simulink model "Tomato_Crop_Control_Main"  (R2025b)
settings: Solver=FixedStepDiscrete  StartTime=0  StopTime=24  FixedStep=0.01  RelTol=1e-3
model workspace (MAT data in the model file):
  Ts = 0.01
  ctrlType = 3
  sensorNoise.time = [0 0.01 0.02 0.03 0.04 0.05 0.06 0.07 0.08 0.09 0.1 0.11 ... (2401 elements, 2401x1)]
  sensorNoise.signals.values = [0.144198042187 -0.535824758394 0.0585721764367 0.102054484425 0.0457535498354 -0.621619945954 0.0176579908891 -0.0995075158765 0.168146871715 0.298844225523 0.375893759453 0.190077020908 ... (26411 elements, 2401x11)]
  sensorNoise.signals.dimensions = 11
  x0 = [60; 25; 65; 15000; 6.35; 2.4; 130; 48; 180; 80; 100]
settings Model: Creator=abhi8  LastModifiedBy=abhi8

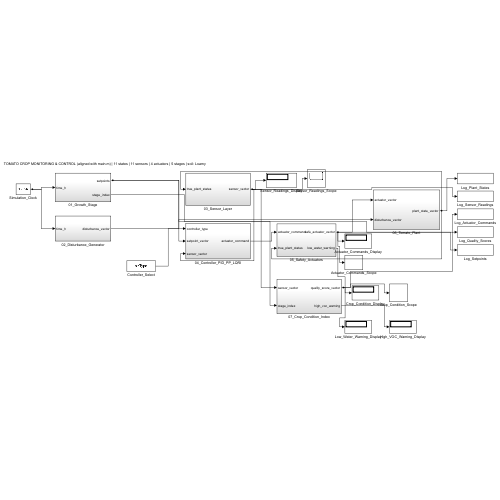
[thumbnail: Simulink's stored preview of the top-level diagram]
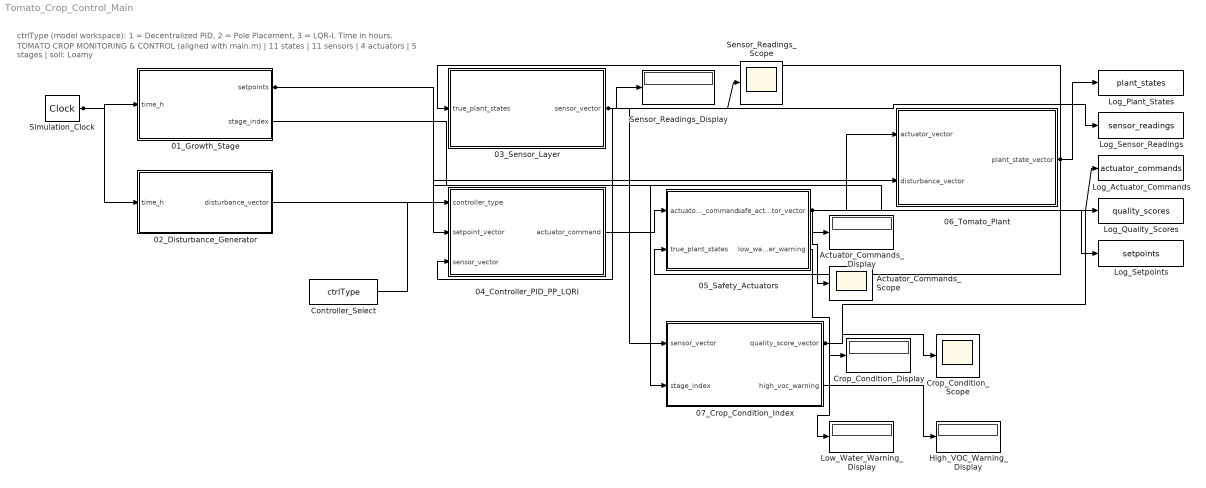
== system Tomato_Crop_Control_Main ==
  note: TOMATO CROP MONITORING & CONTROL (aligned with main.m) | 11 states | 11 sensors | 4 actuators | 5 stages | soil: Loamy
  note: ctrlType (model workspace): 1 = Decentralized PID, 2 = Pole Placement, 3 = LQR-I. Time in hours.
  01_Growth_Stage : Subsystem
  02_Disturbance_Generator : Subsystem
  03_Sensor_Layer : Subsystem
  04_Controller_PID_PP_LQRI : Subsystem
  05_Safety_Actuators : Subsystem
  06_Tomato_Plant : Subsystem
  07_Crop_Condition_Index : Subsystem
  Actuator_Commands_Display : Display
  Actuator_Commands_Scope : Scope
  Controller_Select : Constant  Value=ctrlType  SampleTime=Ts
  Crop_Condition_Display : Display
  Crop_Condition_Scope : Scope
  High_VOC_Warning_Display : Display
  Log_Actuator_Commands : ToWorkspace  VariableName=actuator_commands  SaveFormat=Timeseries  SampleTime=-1
  Log_Plant_States : ToWorkspace  VariableName=plant_states  SaveFormat=Timeseries  SampleTime=-1
  Log_Quality_Scores : ToWorkspace  VariableName=quality_scores  SaveFormat=Timeseries  SampleTime=-1
  Log_Sensor_Readings : ToWorkspace  VariableName=sensor_readings  SaveFormat=Timeseries  SampleTime=-1
  Log_Setpoints : ToWorkspace  VariableName=setpoints  SaveFormat=Timeseries  SampleTime=-1
  Low_Water_Warning_Display : Display
  Sensor_Readings_Display : Display
  Sensor_Readings_Scope : Scope
  Simulation_Clock : DigitalClock  SampleTime=Ts
  wires:
  Simulation_Clock/1 -> 01_Growth_Stage/1(time_h), 02_Disturbance_Generator/1(time_h)
  06_Tomato_Plant/1(plant_state_vector) -> 03_Sensor_Layer/1(true_plant_states), 05_Safety_Actuators/2(true_plant_states), Log_Plant_States/1
  Controller_Select/1 -> 04_Controller_PID_PP_LQRI/1(controller_type)
  01_Growth_Stage/1(setpoints) -> 04_Controller_PID_PP_LQRI/2(setpoint_vector), Log_Setpoints/1
  03_Sensor_Layer/1(sensor_vector) -> 04_Controller_PID_PP_LQRI/3(sensor_vector), 07_Crop_Condition_Index/1(sensor_vector), Sensor_Readings_Display/1, Sensor_Readings_Scope/1, Log_Sensor_Readings/1
  04_Controller_PID_PP_LQRI/1(actuator_command) -> 05_Safety_Actuators/1(actuator_command)
  05_Safety_Actuators/1(safe_actuator_vector) -> 06_Tomato_Plant/1(actuator_vector), Actuator_Commands_Display/1, Actuator_Commands_Scope/1, Log_Actuator_Commands/1
  02_Disturbance_Generator/1(disturbance_vector) -> 06_Tomato_Plant/2(disturbance_vector)
  01_Growth_Stage/2(stage_index) -> 07_Crop_Condition_Index/2(stage_index)
  07_Crop_Condition_Index/1(quality_score_vector) -> Crop_Condition_Display/1, Crop_Condition_Scope/1, Log_Quality_Scores/1
  05_Safety_Actuators/2(low_water_warning) -> Low_Water_Warning_Display/1
  07_Crop_Condition_Index/2(high_voc_warning) -> High_VOC_Warning_Display/1

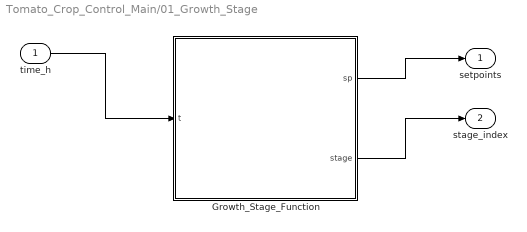
== system Tomato_Crop_Control_Main/01_Growth_Stage ==
  time_h : Inport
  Growth_Stage_Function : MATLAB Function  TreatAsAtomicUnit=on
  setpoints : Outport
  stage_index : Outport  Port=2
  wires:
  time_h/1 -> Growth_Stage_Function/1(t)
  Growth_Stage_Function/1(sp) -> setpoints/1
  Growth_Stage_Function/2(stage) -> stage_index/1

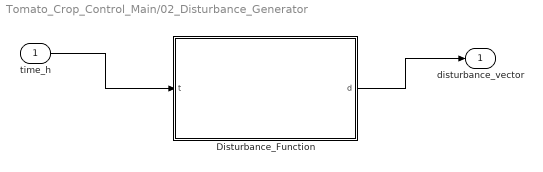
== system Tomato_Crop_Control_Main/02_Disturbance_Generator ==
  time_h : Inport
  Disturbance_Function : MATLAB Function  TreatAsAtomicUnit=on
  disturbance_vector : Outport
  wires:
  time_h/1 -> Disturbance_Function/1(t)
  Disturbance_Function/1(d) -> disturbance_vector/1

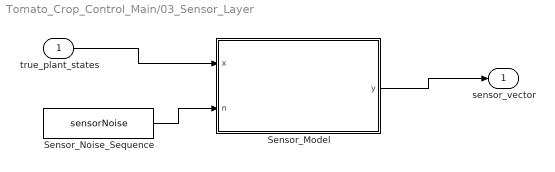
== system Tomato_Crop_Control_Main/03_Sensor_Layer ==
  true_plant_states : Inport
  Sensor_Model : MATLAB Function  TreatAsAtomicUnit=on
  Sensor_Noise_Sequence : FromWorkspace  VariableName=sensorNoise  SampleTime=Ts  Interpolate=off  OutputAfterFinalValue=Holding final value
  sensor_vector : Outport
  wires:
  true_plant_states/1 -> Sensor_Model/1(x)
  Sensor_Noise_Sequence/1 -> Sensor_Model/2(n)
  Sensor_Model/1(y) -> sensor_vector/1

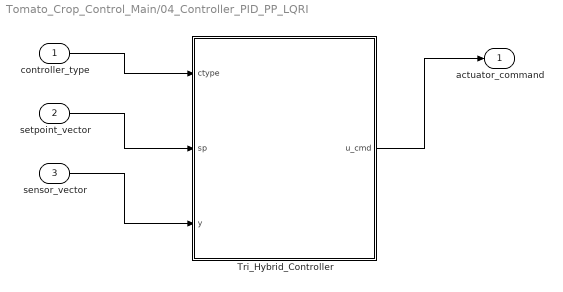
== system Tomato_Crop_Control_Main/04_Controller_PID_PP_LQRI ==
  controller_type : Inport
  setpoint_vector : Inport  Port=2
  sensor_vector : Inport  Port=3
  Tri_Hybrid_Controller : MATLAB Function  TreatAsAtomicUnit=on
  actuator_command : Outport
  wires:
  controller_type/1 -> Tri_Hybrid_Controller/1(ctype)
  setpoint_vector/1 -> Tri_Hybrid_Controller/2(sp)
  sensor_vector/1 -> Tri_Hybrid_Controller/3(y)
  Tri_Hybrid_Controller/1(u_cmd) -> actuator_command/1

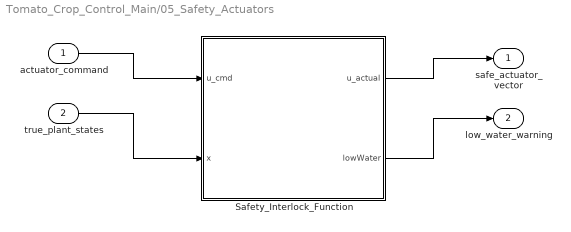
== system Tomato_Crop_Control_Main/05_Safety_Actuators ==
  actuator_command : Inport
  true_plant_states : Inport  Port=2
  Safety_Interlock_Function : MATLAB Function  TreatAsAtomicUnit=on
  safe_actuator_vector : Outport
  low_water_warning : Outport  Port=2
  wires:
  actuator_command/1 -> Safety_Interlock_Function/1(u_cmd)
  true_plant_states/1 -> Safety_Interlock_Function/2(x)
  Safety_Interlock_Function/1(u_actual) -> safe_actuator_vector/1
  Safety_Interlock_Function/2(lowWater) -> low_water_warning/1

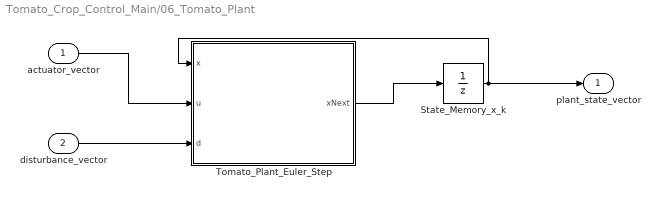
== system Tomato_Crop_Control_Main/06_Tomato_Plant ==
  actuator_vector : Inport
  disturbance_vector : Inport  Port=2
  State_Memory_x_k : UnitDelay  InitialCondition=x0  SampleTime=0.01  HasFrameUpgradeWarning=on
  Tomato_Plant_Euler_Step : MATLAB Function  TreatAsAtomicUnit=on
  plant_state_vector : Outport
  wires:
  State_Memory_x_k/1 -> Tomato_Plant_Euler_Step/1(x), plant_state_vector/1
  actuator_vector/1 -> Tomato_Plant_Euler_Step/2(u)
  disturbance_vector/1 -> Tomato_Plant_Euler_Step/3(d)
  Tomato_Plant_Euler_Step/1(xNext) -> State_Memory_x_k/1

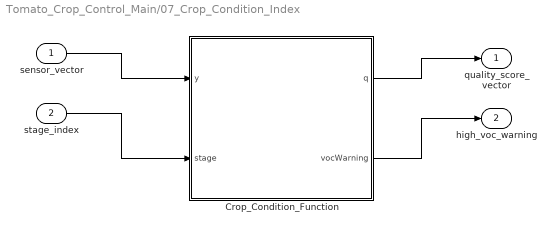
== system Tomato_Crop_Control_Main/07_Crop_Condition_Index ==
  sensor_vector : Inport
  stage_index : Inport  Port=2
  Crop_Condition_Function : MATLAB Function  TreatAsAtomicUnit=on
  quality_score_vector : Outport
  high_voc_warning : Outport  Port=2
  wires:
  sensor_vector/1 -> Crop_Condition_Function/1(y)
  stage_index/1 -> Crop_Condition_Function/2(stage)
  Crop_Condition_Function/1(q) -> quality_score_vector/1
  Crop_Condition_Function/2(vocWarning) -> high_voc_warning/1

== matlab function Tomato_Crop_Control_Main/01_Growth_Stage/Growth_Stage_Function ==
  data: t input; sp output; stage output
function [sp, stage] = GrowthStage(t)
% sp = [moisture; temperature; humidity; light] (main.m db.phase setpoints)
if t < 2
    stage = 1; sp = [70;24;72.5;10000];
elseif t < 8
    stage = 2; sp = [60;25;65;18000];
elseif t < 12
    stage = 3; sp = [58;23.5;62.5;22500];
elseif t < 18
    stage = 4; sp = [65;25;60;22500];
else
    stage = 5; sp = [55;22.5;55;20000];
end
end

== matlab function Tomato_Crop_Control_Main/03_Sensor_Layer/Sensor_Model ==
  data: x input; y output; n input
function y = SensorModel(x, n)
% main.m simulateSensorLayerLocal: y = sat(x + sigma*randn), randn sequence fed in as n
lo = [0;-40;0;0;0;0;0;0;0;0;0];
hi = [100;85;100;65535;14;10;1999;1999;1999;100;500];
noiseOn = 1;
y = zeros(11, 1);
for i = 1:11
    sensed = x(i) + noiseOn * n(i);
    y(i) = max(lo(i), min(hi(i), sensed));
end
end

== matlab function Tomato_Crop_Control_Main/04_Controller_PID_PP_LQRI/Tri_Hybrid_Controller ==
  data: ctype input; u_cmd output; sp input; y input
function u_cmd = TriHybridController(ctype, sp, y)
% ctype: 1 = Decentralized PID, 2 = Pole Placement, 3 = LQR-I (main.m step 6 switch)
persistent intg pe z_int
dt = 0.01;
Kp = [0.080000000000000002;0.20000000000000001;0.10000000000000001;5.0000000000000002e-05];
Ki = [0.014999999999999999;0.02;0.014999999999999999;1.0000000000000001e-05];
Kd = [0.0050000000000000001;0.01;0.0050000000000000001;1.0000000000000001e-05];
u0 = [0.14999999999999999;0.40000000000000008;0.20000000000000004;0];
x0t = [60;25;65;15000;6.3569767441860456;3.0961538461538458;132.14617940199335;53.157370517928278;193.97515527950313;80;100];
Kpp = [0.048333333337184523 -0.00049572649547191604 0 -1.2803268095182857e-08 0 0 0 0 0 0 0;0 -0.21666666660225375 -2.7755575615628914e-17 -1.6507937872024044e-05 0 0 0 0 0 0 0;0 -0.14713541663468468 0.12499999999987499 -1.0615080242334755e-05 0 0 0 0 0 0 0;0 0 0 2.3333327691070732e-05 0 0 0 0 0 0 0];
Kx = [0.33045903239628471 -0.00041190708390725835 1.709435974051306e-05 -2.3561558211869358e-09 -0.00048730567058277003 1.1042346765690718e-05 -4.82261767063196e-07 2.5341090944660356e-06 2.1422647797648958e-06 -2.3389542716528394e-06 7.5156450631499362e-18;0.00012071812895227755 -0.9851642748800985 -0.059883029409090759 -2.6221558787539299e-06 8.2842246792511105e-08 -7.0757158985011595e-06 2.1496635984296123e-07 5.9632600152445188e-07 1.8759197603930526e-07 2.8607042231626474e-09 5.2040316388700277e-21;1.1217806681167034e-05 -0.37126976109372778 0.37426516788265268 -7.6341153907015784e-07 4.7389129263811032e-08 -1.7494050334136512e-06 4.6254791841818205e-08 1.2806484979807713e-07 4.019131706525666e-08 8.3160193500875327e-10 6.8202143908703237e-22;-5.8631339014747203e-06 0.046489321360276642 -0.0053677373840816762 0.00039002337891379279 -1.5258171556508284e-07 4.4013012272865192e-07 -9.19215082032534e-07 -2.6187991014429883e-06 -8.0551413105558905e-07 -8.7458293397006619e-10 -5.1872422376848302e-21];
Kz = [0.63245550435268716 0.0004211622899643958 4.0740750688245492e-05 -7.1243543416210205e-09;0.00020984406328235648 -1.5711911017241582 -0.17357717814678505 4.4155060562703391e-05;6.030330919642846e-06 -0.39163748120451147 0.55605516599390314 2.0221198342119552e-05;-4.6424572517600495e-06 0.097211657880012514 -0.0078367674724567678 0.0012232370229141166];
if isempty(intg),  intg  = zeros(4, 1); end
if isempty(pe),    pe    = zeros(4, 1); end
if isempty(z_int), z_int = zeros(4, 1); end
yv = y(:); spv = sp(:);
u_cmd = zeros(4, 1);
% tracking errors from SENSED values (temperature reversed: fan cools)
e = [spv(1) - yv(1); yv(2) - spv(2); spv(3) - yv(3); spv(4) - yv(4)];
xtarget = x0t; xtarget(1:4) = spv;
if ctype == 1
    for j = 1:4
        ur = Kp(j)*e(j) + Ki(j)*intg(j) + Kd(j)*(e(j) - pe(j))/dt;
        u_cmd(j) = max(0, min(1, ur));
        if ~((ur >= 1 && e(j) > 0) || (ur <= 0 && e(j) < 0))
            intg(j) = intg(j) + e(j) * dt;
        end
        pe(j) = e(j);
    end
elseif ctype == 2
    u_cmd = u0 - Kpp * (yv - xtarget);
else
    u_raw = u0 - Kx * (yv - xtarget) - Kz * z_int;
    u_cmd = max(0, min(1, u_raw));
    y_err = yv(1:4) - spv(1:4);
    for j = 1:4
        push = -Kz(j,j) * y_err(j);
        if ~((u_raw(j) >= 1 && push > 0) || (u_raw(j) <= 0 && push < 0))
            z_int(j) = z_int(j) + y_err(j) * dt;
        end
    end
end
end

== matlab function Tomato_Crop_Control_Main/05_Safety_Actuators/Safety_Interlock_Function ==
  data: u_cmd input; u_actual output; x input; lowWater output
function [u_actual, lowWater] = SafetyLogic(u_cmd, x)
% main.m: actuator saturation, then pump cut-off when TRUE tank level < minimum
u_actual = max(0.0, min(1.0, u_cmd(:)));
lowWater = double(x(10) < 10);
if lowWater > 0
    u_actual(1) = 0.0;
end
end

== matlab function Tomato_Crop_Control_Main/06_Tomato_Plant/Tomato_Plant_Euler_Step ==
  data: x input; u input; xNext output; d input
function xNext = TomatoPlantStep(x, u, d)
% main.m Tomato_Dynamics + forward Euler + enforcePhysicalBoundsLocal
% Soil type: Loamy
dt = 0.01;
minWater = 10;
drainageGain = 0.02; irrigationGain = 12; evapFactor = 2;
drainageThreshold = 50; leachFac = 1;
xv = x(:);
pump      = max(0, min(1, u(1)));
fan       = max(0, min(1, u(2)));
mist      = max(0, min(1, u(3)));
growLight = max(0, min(1, u(4)));
if xv(10) < minWater
    pump = 0.0;
end
extT = d(1); natL = d(2); evap = d(3);
M = xv(1); T = xv(2); L = xv(4); pH = xv(5); EC = xv(6);
N = xv(7); P = xv(8); K = xv(9); VOC = xv(11);
drainage = drainageGain * max(M - drainageThreshold, 0);
moistureLoss = evapFactor * evap * (1 + 0.01 * max(T - 25, 0));
dM = irrigationGain * pump - moistureLoss - drainage;
dT = 0.15 * (extT - T) + 0.00008 * L - 3.0 * fan;
dH = 8.0 * mist - 4.0 * fan - 0.15 * max(T - 25, 0);
dL = 0.5 * (natL - L) + 30000.0 * growLight;
transpiration = (0.50 + 0.50 * (L / 25000.0)) * (1.0 + 0.02 * max(T - 22, 0));
dpH = 0.04 * (6.35 - pH) + 0.02 * (6.45 - pH) * pump - 0.0002 * max(N - 140, 0);
dEC = 0.55 * pump - 0.05 * (evap / 0.8) - 0.03 * leachFac * drainage * EC + 0.02 * (2.4 - EC);
dN = 22.0 * pump - 3.8 * transpiration - 0.05 * leachFac * drainage * (N / 100.0) + 0.03 * (130.0 - N);
dP = 7.5 * pump - 1.2 * transpiration - 0.02 * leachFac * drainage * (P / 50.0) + 0.02 * (48.0 - P);
dK = 28.0 * pump - 4.8 * transpiration - 0.04 * leachFac * drainage * (K / 150.0) + 0.03 * (190.0 - K);
refillNominal = 0.5 * evap + 0.2 * 0.15;
q_refill = 0.05 * (80.0 - xv(10)) + refillNominal;
dWater = q_refill - (0.5 * evap + 0.2 * pump);
dVOC = 0.05 * (100.0 - VOC) + 0.10 * max(T - 30, 0);
dx = [dM; dT; dH; dL; dpH; dEC; dN; dP; dK; dWater; dVOC];
xNext = xv + dx * dt;
lo = [0; -10; 0; 0; 0; 0; 0; 0; 0; 0; 0];
hi = [100; 60; 100; 100000; 14; 15; 500; 500; 500; 100; 500];
xNext = max(lo, min(hi, xNext));
end

== matlab function Tomato_Crop_Control_Main/07_Crop_Condition_Index/Crop_Condition_Function ==
  data: y input; q output; stage input; vocWarning output
function [q, vocWarning] = CropQuality(y, stage)
% main.m calcQualityOnlineLocal; q = [environmental; soil; nutrient; overall]
st = max(1, min(5, round(stage)));
switch st
case 1
    Tr=[20 28]; Hr=[65 80]; Mr=[60 80]; Lr=[5000 15000];
    pHr=[6 6.5999999999999996]; ECr=[1.6000000000000001 2.5]; Nr=[90 140]; Pr=[30 55]; Kr=[120 180];
case 2
    Tr=[21 27]; Hr=[55 75]; Mr=[50 70]; Lr=[12000 25000];
    pHr=[6 6.5999999999999996]; ECr=[1.8 2.7000000000000002]; Nr=[115 165]; Pr=[35 60]; Kr=[140 200];
case 3
    Tr=[20 26]; Hr=[50 70]; Mr=[50 65]; Lr=[15000 30000];
    pHr=[6.0999999999999996 6.7000000000000002]; ECr=[2 2.8999999999999999]; Nr=[110 155]; Pr=[40 68]; Kr=[155 220];
case 4
    Tr=[21 28]; Hr=[50 70]; Mr=[55 75]; Lr=[15000 30000];
    pHr=[6.0999999999999996 6.7000000000000002]; ECr=[2.1000000000000001 3.1000000000000001]; Nr=[105 150]; Pr=[38 62]; Kr=[165 230];
otherwise
    Tr=[18 26]; Hr=[45 65]; Mr=[45 65]; Lr=[12000 28000];
    pHr=[6 6.5999999999999996]; ECr=[2.2000000000000002 3.2000000000000002]; Nr=[95 140]; Pr=[32 55]; Kr=[150 210];
end
qEnv  = (rSc(y(2), Tr(1), Tr(2)) + rSc(y(3), Hr(1), Hr(2)) + rSc(y(1), Mr(1), Mr(2)) + rSc(y(4), Lr(1), Lr(2))) / 4.0;
qSoil = (rSc(y(5), pHr(1), pHr(2)) + rSc(y(6), ECr(1), ECr(2))) / 2.0;
qNutr = (rSc(y(7), Nr(1), Nr(2)) + rSc(y(8), Pr(1), Pr(2)) + rSc(y(9), Kr(1), Kr(2))) / 3.0;
qTot  = max(0, min(100, 0.50 * qEnv + 0.25 * qSoil + 0.25 * qNutr));
q = [qEnv; qSoil; qNutr; qTot];
vocWarning = double(y(11) > 200);   % extra alarm (not part of main.m CCI)
end

function s = rSc(val, low, high)
if val >= low && val <= high
    s = 100.0;
elseif val < low
    s = max(0.0, 100.0 - ((low - val) / max(low * 0.40, 1.0)) * 100.0);
else
    s = max(0.0, 100.0 - ((val - high) / max(high * 0.40, 1.0)) * 100.0);
end
end

== matlab function Tomato_Crop_Control_Main/02_Disturbance_Generator/Disturbance_Function ==
  data: t input; d output
function d = DisturbanceGenerator(t)
% main.m getDisturbancesLocal
t_day = mod(t, 24);
extT = 23.5 + 5.5 * sin(2 * pi * (t_day - 9.5) / 24);
if t_day >= 6.0 && t_day <= 19.5
    natL = max(0, 22000.0 * sin(pi * (t_day - 6.0) / 13.5));
else
    natL = 0.0;
end
evap = 0.35 + 0.60 * (natL / 22000.0) + 0.03 * max(extT - 22.0, 0);
d = [extT; natL; evap];
end
